simulink model "AKident"  (R2026b)
values from neighbouring files (symbols this model uses):
  sigma2v = 0    [zad2_settings.m]    (also in zad3_settings.m = 0.001)
  Tp = 1    [zad2_settings.m]    (also in zad3_settings.m = 0.5)
libraries: simulink x1
settings Model: Creator=Paweł  LastModifiedBy=Paweł

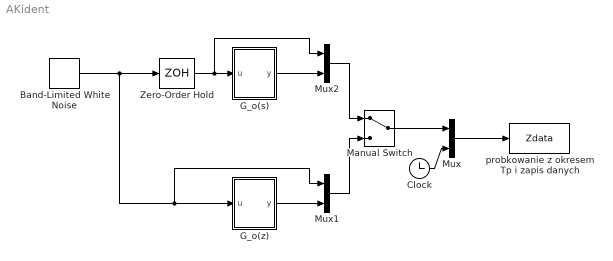
== system AKident ==
  Band-Limited White Noise : simulink/Sources/Band-Limited White Noise  Cov=[0.5]*Tp  Ts=Tp  seed=[23341]
  Clock : Clock
  G_o(s) : Subsystem
  G_o(z) : Subsystem
  Manual Switch : ManualSwitch
  Mux : Mux  Inputs=2
  Mux1 : Mux  Inputs=2
  Mux2 : Mux  Inputs=2
  Zero-Order Hold : ZeroOrderHold  SampleTime=Tp
  probkowanie z okresem Tp i zapis danych : ToWorkspace  VariableName=Zdata  SampleTime=Tp
  wires:
  Zero-Order Hold/1 -> G_o(s)/1(u), Mux2/1
  Band-Limited White Noise/1 -> Zero-Order Hold/1, G_o(z)/1(u), Mux1/1
  Mux/1 -> probkowanie z okresem Tp i zapis danych/1
  Manual Switch/1 -> Mux/1
  Clock/1 -> Mux/2
  Mux1/1 -> Manual Switch/2
  Mux2/1 -> Manual Switch/1
  G_o(s)/1(y) -> Mux2/2
  G_o(z)/1(y) -> Mux1/2

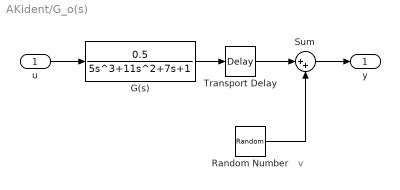
== system AKident/G_o(s) ==
  note: v
  u : Inport
  G(s) : TransferFcn  Numerator=[0.5]  Denominator=[5 11 7 1]
  Random Number : RandomNumber  Variance=sigma2v  Seed=159  SampleTime=Tp*0.1
  Sum : Sum  Inputs=|++
  Transport Delay : TransportDelay  DelayTime=3
  y : Outport
  wires:
  G(s)/1 -> Transport Delay/1
  u/1 -> G(s)/1
  Random Number/1 -> Sum/2
  Sum/1 -> y/1
  Transport Delay/1 -> Sum/1

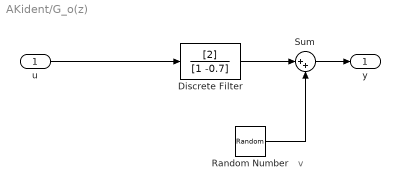
== system AKident/G_o(z) ==
  note: v
  u : Inport
  Discrete Filter : DiscreteFilter  Numerator=[2]  Denominator=[1 -0.7]  SampleTime=Tp
  Random Number : RandomNumber  Variance=sigma2v  Seed=159  SampleTime=Tp
  Sum : Sum  Inputs=|++
  y : Outport
  wires:
  u/1 -> Discrete Filter/1
  Random Number/1 -> Sum/2
  Sum/1 -> y/1
  Discrete Filter/1 -> Sum/1
